simulink model "EightDiscrete"  (R2016a)
settings: Solver=VariableStepAuto  StartTime=0.0  StopTime=100  RelTol=1e-3
undefined symbols (not defined in the file or in its folder): aWS, bWS, DiscIntNeverNeededParam
libraries: simulink x4
settings Model: Creator=kkhan  LastModifiedBy=kkhan

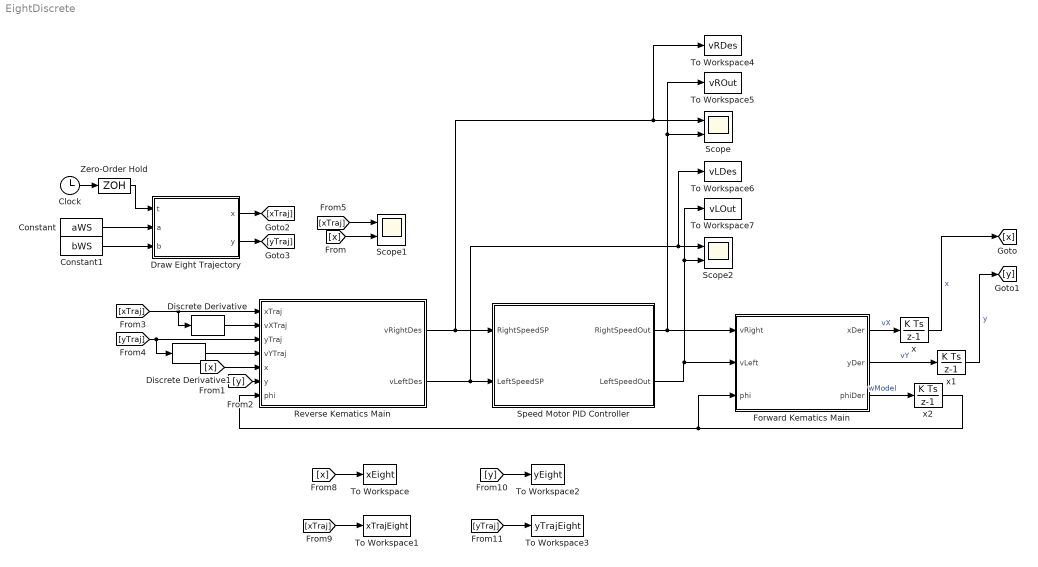
== system EightDiscrete ==
  Clock : Clock
  Constant : Constant  Value=aWS
  Constant1 : Constant  Value=bWS
  Discrete Derivative : simulink/Discrete/Discrete Derivative  gainval=1  ICPrevScaledInput=0  OutMin=[]  OutMax=[]  OutDataType=fixdt(1, 16)  OutScaling=2^-10  DoSatur=off
  Discrete Derivative1 : simulink/Discrete/Discrete Derivative  gainval=1  ICPrevScaledInput=0  OutMin=[]  OutMax=[]  OutDataType=fixdt(1, 16)  OutScaling=2^-10  DoSatur=off
  Draw Eight Trajectory : MATLAB Function  TreatAsAtomicUnit=on
  Forward Kematics Main : MATLAB Function  TreatAsAtomicUnit=on
  Reverse Kematics Main : MATLAB Function  TreatAsAtomicUnit=on
  Scope : Scope  NumInputPorts=2
  Scope1 : Scope  NumInputPorts=2
  Scope2 : Scope  NumInputPorts=2
  Speed Motor PID Controller : Subsystem  TreatAsAtomicUnit=on
  To Workspace : ToWorkspace  VariableName=xEight  SaveFormat=Timeseries  SampleTime=-1
      settings: Decimation=2
  To Workspace1 : ToWorkspace  VariableName=xTrajEight  SaveFormat=Timeseries  SampleTime=-1
      settings: Decimation=2
  To Workspace2 : ToWorkspace  VariableName=yEight  SaveFormat=Timeseries  SampleTime=-1
      settings: Decimation=2
  To Workspace3 : ToWorkspace  VariableName=yTrajEight  SaveFormat=Timeseries  SampleTime=-1
      settings: Decimation=2
  To Workspace4 : ToWorkspace  VariableName=vRDes  SaveFormat=Timeseries  SampleTime=-1
      settings: Decimation=2
  To Workspace5 : ToWorkspace  VariableName=vROut  SaveFormat=Timeseries  SampleTime=-1
      settings: Decimation=2
  To Workspace6 : ToWorkspace  VariableName=vLDes  SaveFormat=Timeseries  SampleTime=-1
      settings: Decimation=2
  To Workspace7 : ToWorkspace  VariableName=vLOut  SaveFormat=Timeseries  SampleTime=-1
      settings: Decimation=2
  Zero-Order Hold : ZeroOrderHold  SampleTime=0.02
  x : DiscreteIntegrator  InitialConditionSetting=State (most efficient)  SampleTime=0.02  ICPrevOutput=DiscIntNeverNeededParam  ICPrevScaledInput=DiscIntNeverNeededParam
  x1 : DiscreteIntegrator  InitialConditionSetting=State (most efficient)  SampleTime=0.02  ICPrevOutput=DiscIntNeverNeededParam  ICPrevScaledInput=DiscIntNeverNeededParam
  x2 : DiscreteIntegrator  InitialConditionSetting=State (most efficient)  SampleTime=0.02  ICPrevOutput=DiscIntNeverNeededParam  ICPrevScaledInput=DiscIntNeverNeededParam
  wires:
  Speed Motor PID Controller/2(LeftSpeedOut) -> To Workspace7/1, Scope2/2, Forward Kematics Main/2(vLeft)
  Forward Kematics Main/1(xDer) -> x/1  "vX"
  Forward Kematics Main/2(yDer) -> x1/1  "vY"
  x/1 -> [x]  "x"
  x1/1 -> [y]  "y"
  Forward Kematics Main/3(phiDer) -> x2/1  "wModel"
  x2/1 -> Reverse Kematics Main/7(phi), Forward Kematics Main/3(phi)
  Discrete Derivative/1 -> Reverse Kematics Main/2(vXTraj)
  Discrete Derivative1/1 -> Reverse Kematics Main/4(vYTraj)
  [x] -> Scope1/2
  [x] -> Reverse Kematics Main/5(x)
  [y] -> Reverse Kematics Main/6(y)
  Draw Eight Trajectory/1(x) -> [xTraj]
  Draw Eight Trajectory/2(y) -> [yTraj]
  [xTraj] -> Discrete Derivative/1, Reverse Kematics Main/1(xTraj)
  [yTraj] -> Discrete Derivative1/1, Reverse Kematics Main/3(yTraj)
  [xTraj] -> Scope1/1
  [x] -> To Workspace/1
  [xTraj] -> To Workspace1/1
  [y] -> To Workspace2/1
  [yTraj] -> To Workspace3/1
  Reverse Kematics Main/1(vRightDes) -> Speed Motor PID Controller/1(RightSpeedSP), To Workspace4/1, Scope/1
  Speed Motor PID Controller/1(RightSpeedOut) -> Forward Kematics Main/1(vRight), Scope/2, To Workspace5/1
  Reverse Kematics Main/2(vLeftDes) -> Speed Motor PID Controller/2(LeftSpeedSP), To Workspace6/1, Scope2/1
  Clock/1 -> Zero-Order Hold/1
  Constant/1 -> Draw Eight Trajectory/2(a)
  Constant1/1 -> Draw Eight Trajectory/3(b)
  Zero-Order Hold/1 -> Draw Eight Trajectory/1(t)

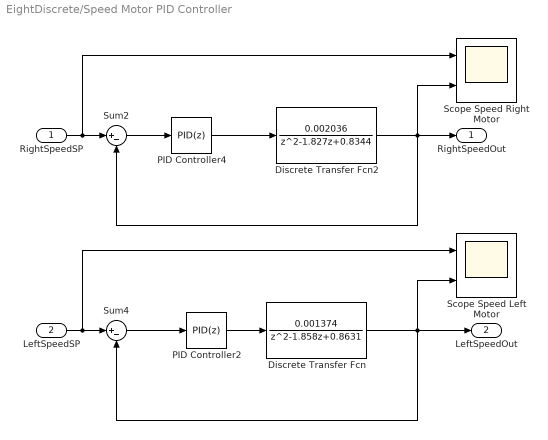
== system EightDiscrete/Speed Motor PID Controller ==
  RightSpeedSP : Inport
  LeftSpeedSP : Inport  Port=2
  Discrete Transfer Fcn : DiscreteTransferFcn  Numerator=[0.001374]  Denominator=[1 -1.858 0.8631]  SampleTime=0.02
  Discrete Transfer Fcn2 : DiscreteTransferFcn  Numerator=[0.002036]  Denominator=[1 -1.827 0.8344]  SampleTime=0.02
  PID Controller2 : simulink/Continuous/PID Controller  Controller=PID  TimeDomain=Discrete-time  SampleTime=0.02  IntegratorMethod=Forward Euler  FilterMethod=Forward Euler  Form=Parallel  UseFilter=on  ControllerParametersSource=internal  P=21.0909852919714  I=43.5478218388463  D=2.15960697462874  N=26.7883535297543  InitialConditionSource=internal  InitialConditionForIntegrator=0  InitialConditionForFilter=0  ExternalReset=none  LimitOutput=off  UpperSaturationLimit=inf  LowerSaturationLimit=-inf  LinearizeAsGain=on  AntiWindupMode=none  Kb=1  TrackingMode=off  Kt=1  PParamMin=[]  PParamMax=[]  IParamMin=[]  IParamMax=[]  DParamMin=[]  DParamMax=[]  NParamMin=[]  NParamMax=[]  KbParamMin=[]  KbParamMax=[]  KtParamMin=[]  KtParamMax=[]  POutMin=[]  POutMax=[]  IOutMin=[]  IOutMax=[]  DOutMin=[]  DOutMax=[]  NOutMin=[]  NOutMax=[]  KbOutMin=[]  KbOutMax=[]  KtOutMin=[]  KtOutMax=[]  IntegratorOutMin=[]  IntegratorOutMax=[]  FilterOutMin=[]  FilterOutMax=[]  SumOutMin=[]  SumOutMax=[]  SumI1OutMin=[]  SumI1OutMax=[]  SumI2OutMin=[]  SumI2OutMax=[]  SumI3OutMin=[]  SumI3OutMax=[]  SumDOutMin=[]  SumDOutMax=[]  SaturationOutMin=[]  SaturationOutMax=[]  IntegratorContinuousStateAttributes=''  IntegratorStateMustResolveToSignalObject=off  IntegratorRTWStateStorageClass=Auto  FilterContinuousStateAttributes=''  FilterStateMustResolveToSignalObject=off  FilterRTWStateStorageClass=Auto  DifferentiatorICPrevScaledInput=0  DifferentiatorOutMin=[]  DifferentiatorOutMax=[]
  PID Controller4 : simulink/Continuous/PID Controller  Controller=PID  TimeDomain=Discrete-time  SampleTime=0.02  IntegratorMethod=Forward Euler  FilterMethod=Forward Euler  Form=Parallel  UseFilter=on  ControllerParametersSource=internal  P=16.8217157087944  I=42.6084644082369  D=1.35986407955998  N=26.7883535297543  InitialConditionSource=internal  InitialConditionForIntegrator=0  InitialConditionForFilter=0  ExternalReset=none  LimitOutput=off  UpperSaturationLimit=inf  LowerSaturationLimit=-inf  LinearizeAsGain=on  AntiWindupMode=none  Kb=1  TrackingMode=off  Kt=1  PParamMin=[]  PParamMax=[]  IParamMin=[]  IParamMax=[]  DParamMin=[]  DParamMax=[]  NParamMin=[]  NParamMax=[]  KbParamMin=[]  KbParamMax=[]  KtParamMin=[]  KtParamMax=[]  POutMin=[]  POutMax=[]  IOutMin=[]  IOutMax=[]  DOutMin=[]  DOutMax=[]  NOutMin=[]  NOutMax=[]  KbOutMin=[]  KbOutMax=[]  KtOutMin=[]  KtOutMax=[]  IntegratorOutMin=[]  IntegratorOutMax=[]  FilterOutMin=[]  FilterOutMax=[]  SumOutMin=[]  SumOutMax=[]  SumI1OutMin=[]  SumI1OutMax=[]  SumI2OutMin=[]  SumI2OutMax=[]  SumI3OutMin=[]  SumI3OutMax=[]  SumDOutMin=[]  SumDOutMax=[]  SaturationOutMin=[]  SaturationOutMax=[]  IntegratorContinuousStateAttributes=''  IntegratorStateMustResolveToSignalObject=off  IntegratorRTWStateStorageClass=Auto  FilterContinuousStateAttributes=''  FilterStateMustResolveToSignalObject=off  FilterRTWStateStorageClass=Auto  DifferentiatorICPrevScaledInput=0  DifferentiatorOutMin=[]  DifferentiatorOutMax=[]
  Scope Speed Left Motor : Scope  NumInputPorts=2
  Scope Speed Right Motor : Scope  NumInputPorts=2
  Sum2 : Sum  Inputs=|+-
  Sum4 : Sum  Inputs=|+-
  RightSpeedOut : Outport
  LeftSpeedOut : Outport  Port=2
  wires:
  RightSpeedSP/1 -> Scope Speed Right Motor/1, Sum2/1
  Discrete Transfer Fcn2/1 -> Scope Speed Right Motor/2, RightSpeedOut/1, Sum2/2
  PID Controller4/1 -> Discrete Transfer Fcn2/1
  LeftSpeedSP/1 -> Scope Speed Left Motor/1, Sum4/1
  Discrete Transfer Fcn/1 -> Scope Speed Left Motor/2, LeftSpeedOut/1, Sum4/2
  Sum4/1 -> PID Controller2/1
  PID Controller2/1 -> Discrete Transfer Fcn/1
  Sum2/1 -> PID Controller4/1

== matlab function EightDiscrete/Forward Kematics Main ==
  data: vRight input; xDer output; vLeft input; yDer output; phiDer output; phi input
function [xDer,yDer,phiDer] = forward(vRight, vLeft, phi)
%#codegen
%Thong so mo hinh
lWheel = 8;
c = 4;
%Input la van toc [cm/s]
vModel = (vRight + vLeft)/2;
%Van toc goc nay la cua mo hinh
wModel = (vRight - vLeft)/(2*lWheel);

vectorMatrix = [cos(phi), -c*sin(phi);
            sin(phi), c*cos(phi);
            0, 1];
velMatrix = [vModel;wModel];

posMatrix = vectorMatrix*velMatrix;

xDer = posMatrix(1);
yDer = posMatrix(2);
phiDer = posMatrix(3);

== matlab function EightDiscrete/Reverse Kematics Main ==
  data: xTraj input; vXTraj input; yTraj input; vYTraj input; x input; y input; vRightDes output; vLeftDes output; phi input
function [vRightDes,vLeftDes] = fcn(xTraj,vXTraj,yTraj,vYTraj,x,y,phi)
%#codegen
L = 16;
c = 4;
lx = 22;
ly = 18;
kx = 1;
ky = 1;
%Input la toa do x, y
%Tu do dao ham se ra van toc dai [cm/s]
stateMatrix = [cos(phi), sin(phi);
               (-1/c)*sin(phi), (1/c)*cos(phi)];
velMatrix = stateMatrix*[vXTraj + lx*tanh((kx/lx)*(xTraj-x));
                         vYTraj + ly*tanh((ky/ly)*(yTraj-y))];

M = [1, L/2; 1, -L/2];
velRLMatrix = M*velMatrix;

vRightDes = velRLMatrix(1);
vLeftDes = velRLMatrix(2);

== matlab function EightDiscrete/Draw Eight Trajectory ==
  data: x output; y output; t input; a input; b input
function [x,y] = eight(t,a,b)
%#codegen
w = pi/16;
x = a*sin(w*t);
y = (b/2)*sin(2*w*t);
